simulink model "homeMobileManipulator"  (R2026a)
settings: Solver=ode4  StartTime=0  StopTime=Inf  FixedStep=cfg.rates.plant  MaxStep=cfg.rates.plant  AbsTol=1e-8
PostLoadFcn:
  | hmmSetup;
InitFcn:
  | hmmInitializeRun(bdroot);
values from neighbouring files (symbols this model uses):
  armJointLimits = zeros(numel(idx.arm), 2)    [hmmSetup.m]
  cfg = app.RunCfg    [HomeMobileManipulatorApp.m]    (also in HomeMobileManipulatorExample.m = params.cfg; hmmSetup.m = hmmConfig(); setupParams.m = data.cfg)
undefined symbols (not defined in the file or in its folder): actionQueueInit, actorNameTable, Angle, apertureMap, armPlanInit, Axis, basePlanInit, Custom, Extent, gray, gripperCoupling, invalidRayHits, movableRegistry, objectTargetInit, perceptionStatusInit, placeTargetInit, Position, robotStateInit, Sim3dSensor
libraries: robotmaniplib x20, robotcorelib x18, simulink x9, sim3dcameralib x6, sim3dgroundtruthsensorlib x4, dspmtrx3 x3, slpidlib x3, sim3dlib x3, hdlsllib x2, robotsim3dlib x1
(part 2 of 6)

== system homeMobileManipulator/Perception/GraspRefinement ==
  CameraFrames : Inport
  TaskRequest : Inport  Port=2
  ObjectTarget : Inport  Port=3
  RobotState : Inport  Port=4
  RefineRequestId : Inport  Port=5
  Refine : TriggerPort  VariantControl=(inherit)  PortDimensions=1
  CoarseTarget : BusSelector  OutputSignals=Position,Extent
  RefineService : MATLAB Function  TreatAsAtomicUnit=on
  SimTime : BusSelector  OutputSignals=Timestamp
  RefinedPosition : Outport
  RefineValid : Outport  Port=2
  RefineStatus : Outport  Port=3
  RefineShift : Outport  Port=4
  ServedRefineId : Outport  Port=5
  RefinedExtent : Outport  Description=THE EXTENT THE DESCENT SHOULD USE: the coarse extent with element 3 replaced by the height THIS FRAME MEASURED, and the coarse extent unchanged on every path that measured nothing. The same depth frame that locates the object top face also reads the support plane under it, so their difference is the object height - measured, with no manifest entry and no assumption. ONLY ELEMENT 3 MOVES, AND THE OTHER TWO ARE NOT A DEFECT WAITING TO BE FIXED: the horizontal extents drive the held-object collision box width and the jaw-aperture gate, and this look measures a top-face plateau, which is not the object silhouette. The height is different - the plateau rise above the support plane IS the height, for any shape. Resolved to a full extent inside hmmRefineService rather than here, so the diagram never has to test a magnitude and a zeros(3,1) can never reach a collision box or a grasp clamp.  Port=6
  wires:
  RefineService/6(RefinedExtent) -> RefinedExtent/1
  RefineService/5(ServedRefineId) -> ServedRefineId/1
  RefineService/4(RefineShift) -> RefineShift/1
  RefineService/2(RefineValid) -> RefineValid/1
  RefineService/1(RefinedPosition) -> RefinedPosition/1
  SimTime/1 -> RefineService/6(simTime)  "<Timestamp>"
  RefineRequestId/1 -> RefineService/5(requestId)
  CoarseTarget/1 -> RefineService/3(coarsePosition)  "<Position>"
  CameraFrames/1 -> RefineService/1(frames)
  RobotState/1 -> SimTime/1
  RefineService/3(RefineStatus) -> RefineStatus/1
  CoarseTarget/2 -> RefineService/4(coarseExtent)  "<Extent>"
  ObjectTarget/1 -> CoarseTarget/1
  TaskRequest/1 -> RefineService/2(task)

== system homeMobileManipulator/Perception/RefinementSelect ==
  ObjectTarget : Inport
  RefineRequestId : Inport  Port=2
  RefinedPosition : Inport  Port=3
  RefineValid : Inport  Port=4
  ServedRefineId : Inport  Port=5
  RefinedExtent : Inport  Port=6
  CoarseGraspPoint : BusSelector  Description=THE FALLBACK ARM OF THE REFINEMENT MERGE. Selects Position alone out of the COARSE ObjectTarget bus, the one Perception reconstructed from the four room cameras, and hands it to RefinedOrCoarse as the value to use when the wrist never got a usable second look. A BusSelector rather than tapping the bus twice downstream because the Switch needs a bare [3 1], and selecting here keeps the coarse-vs-refined choice visible as one three-block chain at root instead of hiding it inside a subsystem.  OutputSignals=Position,Extent
  CurrentRefinementValid : Logic  AllPortsSameDT=off  OutDataTypeStr=boolean
  ObjectTargetRefined : BusAssignment  Description=PUBLISHES THE REFINED GRASP POINT AND THE MEASURED OBJECT SIZE. Assigns Position and Extent and nothing else, so Label, GraspExtent, ActorId and the failure fields stay exactly as Perception sourced them. The wrist refines WHERE the object is and HOW TALL it is, never WHAT it is. Extent joined Position here once the wrist look began measuring the object height from its own depth frame: the same frame that locates the top face reads the support plane under it, and the difference is the height, so MotionPlanning/TargetSelect can aim the jaws at a measured mid-height instead of at a fraction of a manifest entry - or, for an object the manifest does not describe, instead of a flat cfg.percep.extentAssumed guess. ONLY ELEMENT 3 OF THE EXTENT EVER DIFFERS; the horizontal pair is passed through, because a top-face plateau is not the object silhouette. Feeds Manipulator and Gripper, the two consumers that touch the object: the arm plan descends to this point and the capture gate measures from it. TaskPlanner DELIBERATELY KEEPS THE COARSE BUS from Perception instead. It uses Position to form BaseGoalPose, which is solved before the base has driven anywhere and therefore long before the wrist has ever seen the object, so feeding it a point that does not exist yet would be an anachronism, not an improvement. The output signal is named ObjectTargetRefined and logged: hmmRunSummary resolves logged buses BY SIGNAL NAME, so leaving it unnamed made every report, plot and app view show the coarse point while the arm correctly flew to the refined one - a reader scoring the run against the report concluded the second look did nothing.  AssignedSignals=Position,Extent
  RefineRequestMatches : RelationalOperator  Operator===  OutDataTypeStr=boolean  RndMeth=Simplest  InputSameDT=off
  RefinedOrCoarse : Switch  Description=THE WRIST REFINEMENT IS ADVISORY, AND THIS BLOCK IS THE WHOLE REASON IT CAN BE. hmmWristRefine returns the coarse position UNCHANGED on every path that is not STATUS_APPLIED - no frame, no depth, out of range, no top face, a shift past cfg.refine.maxShift - and signals that by clearing RefineValid rather than by returning zeros. So u2 ~= 0 selects the refined point and anything else falls through to the coarse one. Without this switch a failed second look would drive the arm at the origin, which is strictly worse than never looking twice. MEASURED: on the shipped run the refined point cuts the lateral error at the mug body axis from 40.09 mm to 0.99 mm, so the APPLIED branch is worth having and the guarded fallback is what makes it safe to take.  Criteria=u2 ~= 0  SaturateOnIntegerOverflow=off  InputSameDT=off
  RefinedOrCoarseExtent : Switch  Description=THE SECOND ARM OF THE REFINEMENT MERGE, AND IT CARRIES A MEASUREMENT RATHER THAN A CORRECTION. RefinedOrCoarse next door chooses WHERE the object is; this one chooses WHAT SIZE it is. Takes the wrist-measured Extent when RefineValid, the coarse Extent otherwise. The two Switches are deliberately separate blocks on the same gate rather than one wider Switch, because the signals have different widths and because a reader should be able to see that a refinement either replaces both or replaces neither. Gated on RefineValid alone here, the height-is-positive condition having already been applied inside hmmRefineService - so this Switch never has to test a magnitude, and a zero-height Extent cannot reach a collision box or a grasp clamp by way of a sign error in the diagram.  Criteria=u2 ~= 0  SaturateOnIntegerOverflow=off  InputSameDT=off
  ObjectTargetInUse : Outport
  wires:
  ObjectTarget/1 -> ObjectTargetRefined/1, CoarseGraspPoint/1
  RefineRequestId/1 -> RefineRequestMatches/1
  ServedRefineId/1 -> RefineRequestMatches/2
  CoarseGraspPoint/2 -> RefinedOrCoarseExtent/3  "<Extent>"
  RefinedExtent/1 -> RefinedOrCoarseExtent/1
  CurrentRefinementValid/1 -> RefinedOrCoarseExtent/2, RefinedOrCoarse/2  "CurrentRefinementValid"
  RefineRequestMatches/1 -> CurrentRefinementValid/1  "RefineRequestMatches"
  RefineValid/1 -> CurrentRefinementValid/2
  RefinedPosition/1 -> RefinedOrCoarse/1
  CoarseGraspPoint/1 -> RefinedOrCoarse/3  "<Position>"
  RefinedOrCoarse/1 -> ObjectTargetRefined/2
  RefinedOrCoarseExtent/1 -> ObjectTargetRefined/3
  ObjectTargetRefined/1 -> ObjectTargetInUse/1  "ObjectTargetRefined"

== system homeMobileManipulator/Perception/SceneGrounding ==
  CameraFrames : Inport  OutDataTypeStr=Bus: CameraFrame  PortDimensions=5  LatchByDelayingOutsideSignal=on
  TaskRequest : Inport  Port=2  OutDataTypeStr=Bus: TaskRequest  LatchByDelayingOutsideSignal=on
  RobotState : Inport  Port=3  OutDataTypeStr=Bus: RobotState  LatchByDelayingOutsideSignal=on
  MovableRegistry : Inport  Port=4  OutDataTypeStr=Bus: MovableRegistry  LatchByDelayingOutsideSignal=on
  ActiveIndex : Inport  Description=Latch the selected queue index before the perception trigger to break planner feedback. The existing capture delay allows the index to settle before reconstruction.  Port=5  OutDataTypeStr=uint8  LatchByDelayingOutsideSignal=on
  Send : TriggerPort  VariantControl=Variant  PortDimensions=1
  Grounding : Subsystem
  Reconstruction : Subsystem
  SceneMapping : Subsystem
  SimTime : BusSelector  OutputSignals=Timestamp
  ActionQueue : Outport  OutDataTypeStr=Bus: ActionQueue  InitialOutput=actionQueueInit
  ObjectTarget : Outport  Port=2  OutDataTypeStr=Bus: ObjectTarget  InitialOutput=objectTargetInit
  PlaceTarget : Outport  Port=3  OutDataTypeStr=Bus: PlaceTarget  InitialOutput=placeTargetInit
  PerceptionStatus : Outport  Port=4  OutDataTypeStr=Bus: PerceptionStatus  InitialOutput=perceptionStatusInit
  wires:
  CameraFrames/1 -> SceneMapping/1(CameraFrames), Reconstruction/1(CameraFrames), Grounding/1(CameraFrames)
  Grounding/2(PerceptionStatus) -> PerceptionStatus/1
  RobotState/1 -> SceneMapping/2(RobotState), SimTime/1
  TaskRequest/1 -> Grounding/2(TaskRequest)
  MovableRegistry/1 -> Reconstruction/3(MovableRegistry)
  ActiveIndex/1 -> Grounding/4(ActiveIndex)
  Grounding/1(ActionQueue) -> ActionQueue/1, Reconstruction/2(ActionQueue)
  SimTime/1 -> Reconstruction/4(SimTime), Grounding/3(SimTime)  "<Timestamp>"
  Reconstruction/1(ObjectTarget) -> ObjectTarget/1
  Reconstruction/2(PlaceTarget) -> PlaceTarget/1

== system homeMobileManipulator/MobileManipulator/Gripper/ClosureDetect ==
  ApertureCmd : Inport
  Aperture : Inport  Port=2
  DriverAngle : Inport  Port=3
  AbsError : Abs
  ApertureError : Sum  Inputs=+-
  ApertureTol : Constant  Value=cfg.gripper.apertureTol
  AtCommand : RelationalOperator  Operator=<=  OutDataTypeStr=boolean  InputSameDT=off
  DriverMoving : simulink/Logic and Bit Operations/Detect Change  vinit=0  OutDataTypeStr=boolean
      settings: LibrarySourceBlock=|
      | hdlsllib/Logic and Bit
      | Operations/Detect
      | Change
  DriverStopped : Logic  Operator=NOT  IconShape=distinctive  AllPortsSameDT=off  OutDataTypeStr=boolean
  SettledAnd : Logic  IconShape=distinctive  AllPortsSameDT=off  OutDataTypeStr=boolean
  Settled : Outport
  wires:
  DriverStopped/1 -> SettledAnd/2  "DriverStopped"
  ApertureError/1 -> AbsError/1  "ApertureError"
  SettledAnd/1 -> Settled/1
  AbsError/1 -> AtCommand/1  "AbsError"
  ApertureTol/1 -> AtCommand/2
  DriverMoving/1 -> DriverStopped/1
  AtCommand/1 -> SettledAnd/1  "AtCommand"
  ApertureCmd/1 -> ApertureError/1
  Aperture/1 -> ApertureError/2
  DriverAngle/1 -> DriverMoving/1

== system homeMobileManipulator/MobileManipulator/Gripper/GraspCandidate ==
  ObjectTarget : Inport  OutDataTypeStr=Bus: ObjectTarget
  CloseRequested : Inport  Port=2
  ActorSelect : Switch  Criteria=u2 ~= 0
  Candidate : BusCreator  Inputs=5  OutDataTypeStr=Bus: GraspCandidate  NonVirtualBus=on
      settings: InheritFromInputs=off
  CandidateValid : Logic  IconShape=distinctive  AllPortsSameDT=off  OutDataTypeStr=boolean
  HalfHeight : Gain  Description=THE CAPTURE GATE MEASURES TO THE OBJECT'S CENTRE, AND ObjectTarget.Position IS NOT IT. Position is the SUPPORT SURFACE under the object - see the Position contract in hmmReconstructTargets and hmmDefineBuses - so half the sourced height, Extent(3)/2, is what carries it to the centre. A matrix gain rather than a Selector and a scalar gain because the result has to be a [3 1] the Sum below can add to Position without a second reshape: [0 0 0; 0 0 0; 0 0 0.5] annihilates x and y and halves z in one block.  Gain=[0 0 0; 0 0 0; 0 0 0.5]  Multiplication=Matrix(K*u)
  NoActor : Constant  Value=cfg.actor.noneId  OutDataTypeStr=uint8  SampleTime=-1
  ObjSelect : BusSelector  OutputSignals=ActorId,Position,GraspExtent,NumCandidates,Valid,Extent
  ObjectCentre : Sum  Description=WHY THE CENTRE AND NOT THE POINT THE ARM WAS AIMED AT. cfg.grasp.captureRadius is cfg.gripper.maxOpenPos/2 + cfg.grasp.captureMargin - the half jaw stroke plus a margin - so it is a statement about the OBJECT lying inside the volume the jaws sweep, not about how well the servo tracked. Comparing the grasp frame against the commanded grasp point instead would reduce the gate to a tracking check that TrackingMetrics already performs, and would make it blind to the one error it exists to catch. WHAT THIS FIXED. Position was fed to GraspCandidate verbatim, so once the Position contract became the support surface the whole deliberate grasp rise - cfg.grasp.heightFraction*Extent(3) + padDrop(GraspExtent), 66.0 mm on the shipped mug - was charged to the gate as error. WithinCapture measured 66.1 mm against a 62.5 mm radius, InCapture went false, and the close faulted NotGraspable with the tool 0.1 mm from the refined target in xy. It had been passing only because the tool used to sit BELOW the support surface (-16.8 mm on the reference run), which is the defect the grasp-height work removed. WHAT IT COSTS. The gate now spends (heightFraction - 1/2)*Extent(3) + padDrop on the deliberate offset: 21.1 mm for the mug, 39.9 mm for the Bottle, the tallest prop that survives the GraspExtent gate. That leaves 58.8 mm and 48.1 mm of horizontal budget respectively, against a 0.1 mm measured tracking error.
  GraspCandidate : Outport  OutDataTypeStr=Bus: GraspCandidate
  wires:
  ActorSelect/1 -> Candidate/1
  HalfHeight/1 -> ObjectCentre/2  "HalfHeight"
  Candidate/1 -> GraspCandidate/1
  ObjSelect/1 -> ActorSelect/1  "<ActorId>"
  ObjSelect/2 -> ObjectCentre/1  "<Position>"
  ObjectCentre/1 -> Candidate/2  "Position"
  ObjSelect/3 -> Candidate/3  "<GraspExtent>"
  ObjSelect/4 -> Candidate/4  "<NumCandidates>"
  ObjSelect/5 -> CandidateValid/1  "<Valid>"
  ObjSelect/6 -> HalfHeight/1  "<Extent>"
  NoActor/1 -> ActorSelect/3
  ObjectTarget/1 -> ObjSelect/1
  CloseRequested/1 -> CandidateValid/2
  CandidateValid/1 -> ActorSelect/2, Candidate/5  "Valid"

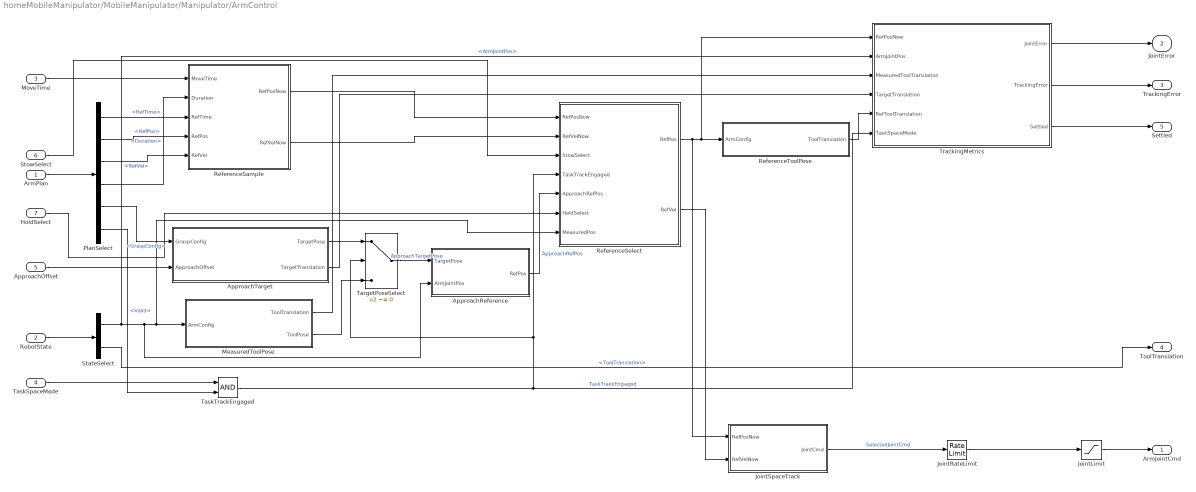
== system homeMobileManipulator/MobileManipulator/Manipulator/ArmControl ==
  ArmPlan : Inport
  RobotState : Inport  Port=2
  MoveTime : Inport  Port=3
  TaskSpaceMode : Inport  Port=4
  ApproachOffset : Inport  Port=5
  StowSelect : Inport  Port=6
  HoldSelect : Inport  Port=7
  ApproachReference : Subsystem  Description=|
      | The joint REFERENCE for a constrained approach or retreat, solved by inverse kinematics that is SEEDED WITH THE MEASURED CONFIGURATION.
      | 
      | WHY THIS EXISTS, AND WHAT IT REPLACES. ArmControl used to carry a second tracker - a Task Space Motion Model - and ModeSelect switched the joint COMMAND between it and JointSpaceTrack on TaskTrackEngaged. Both motion models integrate their own configuration from cfg.arm.stowConfig at t = 0, always, and nothing ever reconciled them. Feeding the task-space model the MEASURED TOOL POSE while it was disengaged was an attempt at bumpless transfer, and it cannot work: a tool pose does not determine a configuration. Measured on the 20 s run, the task-space model free-ran for 6.8 s and settled on a different IK branch - elbow sign-flipped and wrist-3 off by very nearly pi - 4.467 rad from where the arm actually was. ModeSelect handed that branch to JointRateLimit, which ramped toward it at cfg.arm.jointVelMax, the tool error passed cfg.safety.trackErrMax 0.15 s later, and Retreating's tracking guard reported ArmPlanFailed for a plan that had been tracked to 3.4 mm.
      | 
      | SO THERE IS NOW ONE INTEGRATOR. JointSpaceTrack is the only tracker; approach and retreat produce a REFERENCE for it instead of a competing command. TargetPoseSelect is kept and still feeds the approach target when engaged and the measured tool pose when not, but it now feeds an IK solve rather than a motion model - and THE SEED IS WHAT MAKES THAT SOUND. Seeding with the measured configuration pins the solution to the branch the arm is already on, so at the instant of engagement the target is the grasp pose at zero offset, the seed is the current configuration, and the answer is the current configuration. Continuity is a property of the construction rather than something to be hoped for.
  ApproachTarget : Subsystem
  JointLimit : Saturate  UpperLimit=armJointLimits(:,2)  LowerLimit=armJointLimits(:,1)
  JointRateLimit : RateLimiter  RisingSlewLimit=cfg.arm.jointVelMax'  FallingSlewLimit=-cfg.arm.jointVelMax'  SampleTimeMode=inherited  InitialCondition=cfg.arm.stowConfig'
  JointSpaceTrack : Subsystem
  MeasuredToolPose : Subsystem
  PlanSelect : BusSelector  OutputSignals=RefTime,RefPos,RefVel,Duration,GraspConfig,Valid
  ReferenceSample : Subsystem
  ReferenceSelect : Subsystem
  ReferenceToolPose : Subsystem
  StateSelect : BusSelector  OutputSignals=ArmJointPos,ToolTranslation
  TargetPoseSelect : Switch  Description=|  Criteria=u2 ~= 0
      | Approach target when engaged, measured tool pose when not.
      | 
      | Kept from the design this replaces, because the intent was right: the branch that is not in control must be commanded to where the arm IS, so that engaging it is not a step. What changed is the consumer. Handing this to a Task Space Motion Model did not work, because that block integrates its own configuration and a pose does not determine one. Handing it to an IK solve seeded with the measured configuration does.
  TaskTrackEngaged : Logic  Description=The task-space tracker is engaged only when the supervisor asks for task-space mode AND the plan it would chase is valid. Both halves are load-bearing. Without the mode term the tracker integrates through every phase of the task; without the Valid term it chases a GraspConfig that is all zeros when planning failed, which for a UR5e is the fully outstretched singular pose, and the operational-space gains are meaningless there.  AllPortsSameDT=off  OutDataTypeStr=boolean
  TrackingMetrics : Subsystem
  ArmJointCmd : Outport
  JointError : Outport  Port=2
  TrackingError : Outport  Port=3
  ToolTranslation : Outport  Port=4
  Settled : Outport  Port=5
  wires:
  JointRateLimit/1 -> JointLimit/1
  TrackingMetrics/2(TrackingError) -> TrackingError/1
  TrackingMetrics/1(JointError) -> JointError/1
  JointSpaceTrack/1(JointCmd) -> JointRateLimit/1  "SelectedJointCmd"
  ReferenceSelect/2(RefVel) -> JointSpaceTrack/2(RefVelNow)
  ReferenceSelect/1(RefPos) -> ReferenceToolPose/1(ArmConfig), TrackingMetrics/1(RefPosNow), JointSpaceTrack/1(RefPosNow)
  HoldSelect/1 -> ReferenceSelect/6(HoldSelect)
  ApproachReference/1(RefPos) -> ReferenceSelect/5(ApproachRefPos)  "ApproachRefPos"
  TargetPoseSelect/1 -> ApproachReference/1(TargetPose)  "ApproachTargetPose"
  MeasuredToolPose/2(ToolPose) -> TargetPoseSelect/3
  MeasuredToolPose/1(ToolTranslation) -> TrackingMetrics/3(MeasuredToolTranslation)
  ApproachTarget/2(TargetTranslation) -> TrackingMetrics/4(TargetTranslation)
  ApproachTarget/1(TargetPose) -> TargetPoseSelect/1
  ReferenceSample/2(RefVelNow) -> ReferenceSelect/2(RefVelNow)
  ReferenceSample/1(RefPosNow) -> ReferenceSelect/1(RefPosNow)
  TaskSpaceMode/1 -> TaskTrackEngaged/1
  StateSelect/2 -> ToolTranslation/1  "<ToolTranslation>"
  StateSelect/1 -> MeasuredToolPose/1(ArmConfig), ReferenceSelect/7(MeasuredPos), ApproachReference/2(ArmJointPos), TrackingMetrics/2(ArmJointPos)  "<ArmJointPos>"
  JointLimit/1 -> ArmJointCmd/1
  PlanSelect/6 -> TaskTrackEngaged/2  "<Valid>"
  ReferenceToolPose/1(ToolTranslation) -> TrackingMetrics/5(RefToolTranslation)
  TrackingMetrics/3(Settled) -> Settled/1
  PlanSelect/4 -> ReferenceSample/2(Duration)  "<Duration>"
  TaskTrackEngaged/1 -> ReferenceSelect/4(TaskTrackEngaged), TargetPoseSelect/2, TrackingMetrics/6(TaskSpaceMode)  "TaskTrackEngaged"
  PlanSelect/3 -> ReferenceSample/5(RefVel)  "<RefVel>"
  PlanSelect/2 -> ReferenceSample/4(RefPos)  "<RefPos>"
  PlanSelect/1 -> ReferenceSample/3(RefTime)  "<RefTime>"
  PlanSelect/5 -> ApproachTarget/1(GraspConfig)  "<GraspConfig>"
  ArmPlan/1 -> PlanSelect/1
  ApproachOffset/1 -> ApproachTarget/2(ApproachOffset)
  RobotState/1 -> StateSelect/1
  StowSelect/1 -> ReferenceSelect/3(StowSelect)
  MoveTime/1 -> ReferenceSample/1(MoveTime)

== system homeMobileManipulator/MobileManipulator/Manipulator/MotionPlanning ==
  RequestId : Inport  OutDataTypeStr=uint32
  ObjectTarget : Inport  Port=2  OutDataTypeStr=Bus: ObjectTarget
  PlaceTarget : Inport  Port=3  OutDataTypeStr=Bus: PlaceTarget
  RobotState : Inport  Port=4  OutDataTypeStr=Bus: RobotState
  ArmMode : Inport  Port=5  OutDataTypeStr=uint8
  Enable : EnablePort  StatesWhenEnabling=reset
  CandidateIK : Subsystem
  ConfigAssembly : Subsystem
  MapToArmFrame : robotmaniplib/Get Transform  RigidBodyTree=robot  SourceBody=map  TargetBody=arm_mount  SimulateUsing=Code generation
  PrevPlan : UnitDelay  InitialCondition=armPlanInit  SampleTime=-1
  ScreenAndPlan : MATLAB Function  Description=SIMULINK-FIRST JUSTIFICATION: no block in any installed library screens grasp candidates, searches with manipulatorRRT and parameterises with contopptraj. (a) No dedicated toolbox block: find_system('robotmaniplib','SearchDepth',2,'Type','Block') returns 10 blocks - Forward Dynamics, Get Jacobian, Get Transform, Gravity Torque, Inverse Dynamics, Inverse Kinematics, Joint Space Mass Matrix, Joint Space Motion Model, Task Space Motion Model, Velocity Product Torque - and not one of them is a path planner, a collision checker or a time-optimal parameteriser. The four that DO cover part of this job are used as blocks: three Inverse Kinematics, three Get Jacobian, one Get Transform, three Reciprocal Condition. (b) No native Simulink equivalent: manipulatorRRT, checkCollision and contopptraj have no primitive composition - a sampling-based tree search is not a block diagram. (c) The native equivalent is not merely over 15 blocks, it does not exist. Called through coder.extrinsic; the model stays in normal mode.  TreatAsAtomicUnit=on
  SimTime : BusSelector  OutputSignals=Timestamp
  TargetSelect : Subsystem
  ArmPlan : Outport  OutDataTypeStr=Bus: ArmPlan  InitialOutput=armPlanInit
  wires:
  PrevPlan/1 -> ScreenAndPlan/12(planTemplate)
  RequestId/1 -> ScreenAndPlan/10(requestId)
  ScreenAndPlan/1(aplan) -> ArmPlan/1, PrevPlan/1
  CandidateIK/4(GraspPoses) -> ScreenAndPlan/9(graspPoses)
  CandidateIK/3(Manipulability) -> ScreenAndPlan/8(manipulability)
  CandidateIK/2(PoseErrors) -> ScreenAndPlan/7(poseErrors)
  CandidateIK/1(GraspConfigs) -> ScreenAndPlan/6(graspConfigs)
  SimTime/1 -> ScreenAndPlan/11(simTime)  "<Timestamp>"
  MapToArmFrame/1 -> CandidateIK/2(TfArmFromMap), ScreenAndPlan/5(tfArmFromMap)
  ConfigAssembly/2(IkGuess) -> CandidateIK/3(IkGuess)
  ConfigAssembly/1(RobotConfig) -> MapToArmFrame/1, ScreenAndPlan/4(robotConfig)
  PlaceTarget/1 -> TargetSelect/2(PlaceTarget), ScreenAndPlan/2(placeTarget)
  ArmMode/1 -> ScreenAndPlan/3(mode), TargetSelect/3(ArmMode)
  RobotState/1 -> ConfigAssembly/1(RobotState), SimTime/1
  ObjectTarget/1 -> TargetSelect/1(ObjectTarget), ScreenAndPlan/1(objectTarget)
  TargetSelect/1(GraspPoint) -> CandidateIK/1(GraspPoint)

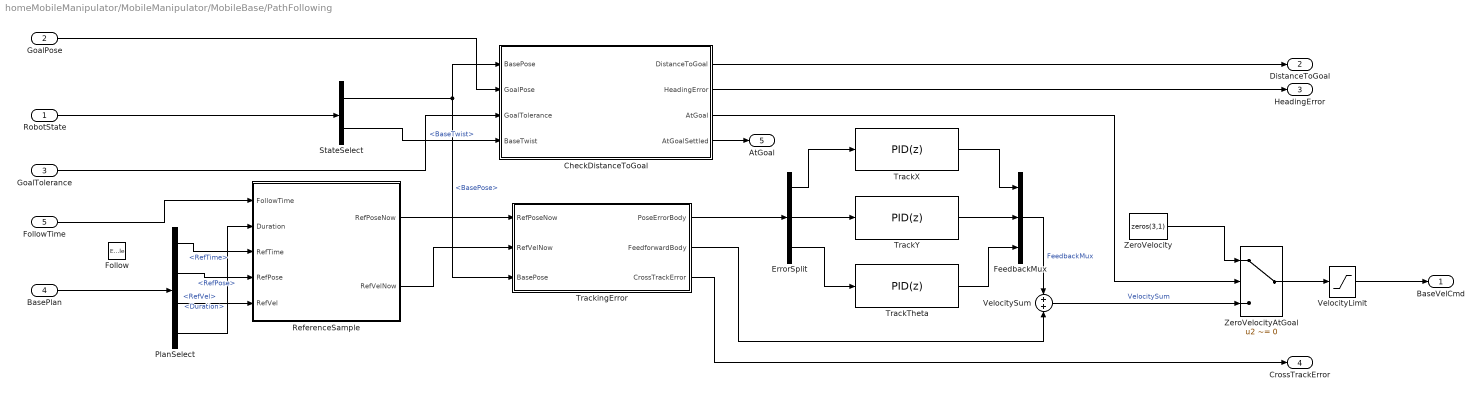
== system homeMobileManipulator/MobileManipulator/MobileBase/PathFollowing ==
  RobotState : Inport
  GoalPose : Inport  Port=2
  GoalTolerance : Inport  Port=3
  BasePlan : Inport  Port=4
  FollowTime : Inport  Port=5
  Follow : EnablePort  StatesWhenEnabling=reset
  CheckDistanceToGoal : Subsystem
  ErrorSplit : Demux  Outputs=3
  FeedbackMux : Mux  Inputs=3
  PlanSelect : BusSelector  OutputSignals=RefTime,RefPose,RefVel,Duration
  ReferenceSample : Subsystem
  StateSelect : BusSelector  OutputSignals=BasePose,BaseTwist
  TrackTheta : slpidlib/PID Controller  Controller=PID  Form=Parallel  TimeDomain=Discrete-time  UseExternalTs=off  SampleTime=cfg.rates.control  IntegratorMethod=Trapezoidal  FilterMethod=Forward Euler  ControllerParametersSource=internal  P=cfg.track.kpTheta  I=cfg.track.kiTheta  UseKiTs=off  D=cfg.track.kdTheta  UseExternalDerivativeSource=off  N=100  UseFilter=on  TunerSelectOption=Transfer Function Based (PID Tuner App)  InitialConditionSource=internal  InitialConditionForIntegrator=0  InitialConditionForFilter=0  DifferentiatorICPrevScaledInput=0  ExternalReset=none  TrackingMode=off  Kt=1  LimitOutput=on  SatLimitsSource=internal  UpperSaturationLimit=cfg.base.omegaMax  LowerSaturationLimit=-cfg.base.omegaMax  LinearizeAsGain=off  AntiWindupMode=clamping  Kb=1  LimitIntegrator=off  UpperIntegratorSaturationLimit=inf  LowerIntegratorSaturationLimit=-inf  POutMin=[]  POutMax=[]  IOutMin=[]  IOutMax=[]  DOutMin=[]  DOutMax=[]  NOutMin=[]  NOutMax=[]  SumOutMin=[]  SumOutMax=[]  SaturationOutMin=[]  SaturationOutMax=[]  PParamMin=[]  PParamMax=[]  IParamMin=[]  IParamMax=[]  DParamMin=[]  DParamMax=[]  NParamMin=[]  NParamMax=[]  KbParamMin=[]  KbParamMax=[]  KtParamMin=[]  KtParamMax=[]  KbOutMin=[]  KbOutMax=[]  KtOutMin=[]  KtOutMax=[]  IntegratorOutMin=[]  IntegratorOutMax=[]  FilterOutMin=[]  FilterOutMax=[]  SumI1OutMin=[]  SumI1OutMax=[]  SumI2OutMin=[]  SumI2OutMax=[]  SumI3OutMin=[]  SumI3OutMax=[]  SumI4OutMin=[]  SumI4OutMax=[]  SumDOutMin=[]  SumDOutMax=[]  DifferentiatorOutMin=[]  DifferentiatorOutMax=[]  FilterDiffOutCoefMin=[]  FilterDiffOutCoefMax=[]  ReciprocalOutMin=[]  ReciprocalOutMax=[]  SumDenOutMin=[]  SumDenOutMax=[]  SumNumOutMin=[]  SumNumOutMax=[]  DivideOutMin=[]  DivideOutMax=[]  UdiffTsProdOutMin=[]  UdiffTsProdOutMax=[]  NTsProdOutMin=[]  NTsProdOutMax=[]  UintegralTsProdOutMin=[]  UintegralTsProdOutMax=[]  UngainTsProdOutMin=[]  UngainTsProdOutMax=[]  ClampingZeroOutDataTypeStr=Inherit: Inherit via back propagation  ClampingZeroOutMin=[]  ClampingZeroOutMax=[]  FilterDenConstantOutDataTypeStr=Inherit: Inherit via back propagation  FilterDenConstantOutMin=[]  FilterDenConstantOutMax=[]  PCopyOutDataTypeStr=Inherit: Inherit via back propagation  PCopyOutMin=[]  PCopyOutMax=[]  NCopyOutDataTypeStr=Inherit: Inherit via back propagation  NCopyOutMin=[]  NCopyOutMax=[]  IntegratorContinuousStateAttributes=''  IntegratorStateMustResolveToSignalObject=off  IntegratorRTWStateStorageClass=Auto  FilterContinuousStateAttributes=''  FilterStateMustResolveToSignalObject=off  FilterRTWStateStorageClass=Auto  ParallelPVariant=InternalParameters  IdealPVariant=Disabled  IVariant=InternalParameters  DVariant=InternalParameters  IntegratorVariant=Discrete  SatVariant=Enabled  AWVariant=DiscClampingParallel  PCopyVariant=Disabled  TRVariant=Disabled  FdbkBlocksVariant=Feedback  IdealPFdbkVariant=Passthrough  SatFdbkVariant=Passthrough  DerivativeFilterVariant=ForwardEulerFilter  NVariant=InternalParameters  NCopyVariant=Disabled  FilterICVariant=InternalICsFilter  IntegratorICVariant=InternalICs  ExternalResetVariant=Disabled  TRSumVariant=Passthrough  SumFdbkVariant=Enabled  SumVariant=Sum_PID  TsampFilterVariant=InternalTs  TsampNgainVariant=Passthrough  TsampIntegralVariant=Disabled_SignalSpec  ExternalSaturationOutDataTypeStr=Inherit: Same as second input  DerivativeSourceVariant=ErrorSignal  PreIntVariant=InternalPreInt
      settings: LibrarySourceBlock=simulink/Discrete/Discrete PID Controller
  TrackX : slpidlib/PID Controller  Controller=PID  Form=Parallel  TimeDomain=Discrete-time  UseExternalTs=off  SampleTime=cfg.rates.control  IntegratorMethod=Trapezoidal  FilterMethod=Forward Euler  ControllerParametersSource=internal  P=cfg.track.kpXY  I=cfg.track.kiXY  UseKiTs=off  D=cfg.track.kdXY  UseExternalDerivativeSource=off  N=100  UseFilter=on  TunerSelectOption=Transfer Function Based (PID Tuner App)  InitialConditionSource=internal  InitialConditionForIntegrator=0  InitialConditionForFilter=0  DifferentiatorICPrevScaledInput=0  ExternalReset=none  TrackingMode=off  Kt=1  LimitOutput=on  SatLimitsSource=internal  UpperSaturationLimit=cfg.base.vxMax  LowerSaturationLimit=-cfg.base.vxMax  LinearizeAsGain=off  AntiWindupMode=clamping  Kb=1  LimitIntegrator=off  UpperIntegratorSaturationLimit=inf  LowerIntegratorSaturationLimit=-inf  POutMin=[]  POutMax=[]  IOutMin=[]  IOutMax=[]  DOutMin=[]  DOutMax=[]  NOutMin=[]  NOutMax=[]  SumOutMin=[]  SumOutMax=[]  SaturationOutMin=[]  SaturationOutMax=[]  PParamMin=[]  PParamMax=[]  IParamMin=[]  IParamMax=[]  DParamMin=[]  DParamMax=[]  NParamMin=[]  NParamMax=[]  KbParamMin=[]  KbParamMax=[]  KtParamMin=[]  KtParamMax=[]  KbOutMin=[]  KbOutMax=[]  KtOutMin=[]  KtOutMax=[]  IntegratorOutMin=[]  IntegratorOutMax=[]  FilterOutMin=[]  FilterOutMax=[]  SumI1OutMin=[]  SumI1OutMax=[]  SumI2OutMin=[]  SumI2OutMax=[]  SumI3OutMin=[]  SumI3OutMax=[]  SumI4OutMin=[]  SumI4OutMax=[]  SumDOutMin=[]  SumDOutMax=[]  DifferentiatorOutMin=[]  DifferentiatorOutMax=[]  FilterDiffOutCoefMin=[]  FilterDiffOutCoefMax=[]  ReciprocalOutMin=[]  ReciprocalOutMax=[]  SumDenOutMin=[]  SumDenOutMax=[]  SumNumOutMin=[]  SumNumOutMax=[]  DivideOutMin=[]  DivideOutMax=[]  UdiffTsProdOutMin=[]  UdiffTsProdOutMax=[]  NTsProdOutMin=[]  NTsProdOutMax=[]  UintegralTsProdOutMin=[]  UintegralTsProdOutMax=[]  UngainTsProdOutMin=[]  UngainTsProdOutMax=[]  ClampingZeroOutDataTypeStr=Inherit: Inherit via back propagation  ClampingZeroOutMin=[]  ClampingZeroOutMax=[]  FilterDenConstantOutDataTypeStr=Inherit: Inherit via back propagation  FilterDenConstantOutMin=[]  FilterDenConstantOutMax=[]  PCopyOutDataTypeStr=Inherit: Inherit via back propagation  PCopyOutMin=[]  PCopyOutMax=[]  NCopyOutDataTypeStr=Inherit: Inherit via back propagation  NCopyOutMin=[]  NCopyOutMax=[]  IntegratorContinuousStateAttributes=''  IntegratorStateMustResolveToSignalObject=off  IntegratorRTWStateStorageClass=Auto  FilterContinuousStateAttributes=''  FilterStateMustResolveToSignalObject=off  FilterRTWStateStorageClass=Auto  ParallelPVariant=InternalParameters  IdealPVariant=Disabled  IVariant=InternalParameters  DVariant=InternalParameters  IntegratorVariant=Discrete  SatVariant=Enabled  AWVariant=DiscClampingParallel  PCopyVariant=Disabled  TRVariant=Disabled  FdbkBlocksVariant=Feedback  IdealPFdbkVariant=Passthrough  SatFdbkVariant=Passthrough  DerivativeFilterVariant=ForwardEulerFilter  NVariant=InternalParameters  NCopyVariant=Disabled  FilterICVariant=InternalICsFilter  IntegratorICVariant=InternalICs  ExternalResetVariant=Disabled  TRSumVariant=Passthrough  SumFdbkVariant=Enabled  SumVariant=Sum_PID  TsampFilterVariant=InternalTs  TsampNgainVariant=Passthrough  TsampIntegralVariant=Disabled_SignalSpec  ExternalSaturationOutDataTypeStr=Inherit: Same as second input  DerivativeSourceVariant=ErrorSignal  PreIntVariant=InternalPreInt
      settings: LibrarySourceBlock=simulink/Discrete/Discrete PID Controller
  TrackY : slpidlib/PID Controller  Controller=PID  Form=Parallel  TimeDomain=Discrete-time  UseExternalTs=off  SampleTime=cfg.rates.control  IntegratorMethod=Trapezoidal  FilterMethod=Forward Euler  ControllerParametersSource=internal  P=cfg.track.kpXY  I=cfg.track.kiXY  UseKiTs=off  D=cfg.track.kdXY  UseExternalDerivativeSource=off  N=100  UseFilter=on  TunerSelectOption=Transfer Function Based (PID Tuner App)  InitialConditionSource=internal  InitialConditionForIntegrator=0  InitialConditionForFilter=0  DifferentiatorICPrevScaledInput=0  ExternalReset=none  TrackingMode=off  Kt=1  LimitOutput=on  SatLimitsSource=internal  UpperSaturationLimit=cfg.base.vyMax  LowerSaturationLimit=-cfg.base.vyMax  LinearizeAsGain=off  AntiWindupMode=clamping  Kb=1  LimitIntegrator=off  UpperIntegratorSaturationLimit=inf  LowerIntegratorSaturationLimit=-inf  POutMin=[]  POutMax=[]  IOutMin=[]  IOutMax=[]  DOutMin=[]  DOutMax=[]  NOutMin=[]  NOutMax=[]  SumOutMin=[]  SumOutMax=[]  SaturationOutMin=[]  SaturationOutMax=[]  PParamMin=[]  PParamMax=[]  IParamMin=[]  IParamMax=[]  DParamMin=[]  DParamMax=[]  NParamMin=[]  NParamMax=[]  KbParamMin=[]  KbParamMax=[]  KtParamMin=[]  KtParamMax=[]  KbOutMin=[]  KbOutMax=[]  KtOutMin=[]  KtOutMax=[]  IntegratorOutMin=[]  IntegratorOutMax=[]  FilterOutMin=[]  FilterOutMax=[]  SumI1OutMin=[]  SumI1OutMax=[]  SumI2OutMin=[]  SumI2OutMax=[]  SumI3OutMin=[]  SumI3OutMax=[]  SumI4OutMin=[]  SumI4OutMax=[]  SumDOutMin=[]  SumDOutMax=[]  DifferentiatorOutMin=[]  DifferentiatorOutMax=[]  FilterDiffOutCoefMin=[]  FilterDiffOutCoefMax=[]  ReciprocalOutMin=[]  ReciprocalOutMax=[]  SumDenOutMin=[]  SumDenOutMax=[]  SumNumOutMin=[]  SumNumOutMax=[]  DivideOutMin=[]  DivideOutMax=[]  UdiffTsProdOutMin=[]  UdiffTsProdOutMax=[]  NTsProdOutMin=[]  NTsProdOutMax=[]  UintegralTsProdOutMin=[]  UintegralTsProdOutMax=[]  UngainTsProdOutMin=[]  UngainTsProdOutMax=[]  ClampingZeroOutDataTypeStr=Inherit: Inherit via back propagation  ClampingZeroOutMin=[]  ClampingZeroOutMax=[]  FilterDenConstantOutDataTypeStr=Inherit: Inherit via back propagation  FilterDenConstantOutMin=[]  FilterDenConstantOutMax=[]  PCopyOutDataTypeStr=Inherit: Inherit via back propagation  PCopyOutMin=[]  PCopyOutMax=[]  NCopyOutDataTypeStr=Inherit: Inherit via back propagation  NCopyOutMin=[]  NCopyOutMax=[]  IntegratorContinuousStateAttributes=''  IntegratorStateMustResolveToSignalObject=off  IntegratorRTWStateStorageClass=Auto  FilterContinuousStateAttributes=''  FilterStateMustResolveToSignalObject=off  FilterRTWStateStorageClass=Auto  ParallelPVariant=InternalParameters  IdealPVariant=Disabled  IVariant=InternalParameters  DVariant=InternalParameters  IntegratorVariant=Discrete  SatVariant=Enabled  AWVariant=DiscClampingParallel  PCopyVariant=Disabled  TRVariant=Disabled  FdbkBlocksVariant=Feedback  IdealPFdbkVariant=Passthrough  SatFdbkVariant=Passthrough  DerivativeFilterVariant=ForwardEulerFilter  NVariant=InternalParameters  NCopyVariant=Disabled  FilterICVariant=InternalICsFilter  IntegratorICVariant=InternalICs  ExternalResetVariant=Disabled  TRSumVariant=Passthrough  SumFdbkVariant=Enabled  SumVariant=Sum_PID  TsampFilterVariant=InternalTs  TsampNgainVariant=Passthrough  TsampIntegralVariant=Disabled_SignalSpec  ExternalSaturationOutDataTypeStr=Inherit: Same as second input  DerivativeSourceVariant=ErrorSignal  PreIntVariant=InternalPreInt
      settings: LibrarySourceBlock=simulink/Discrete/Discrete PID Controller
  TrackingError : Subsystem
  VelocityLimit : Saturate  UpperLimit=cfg.base.cmdMargin*[cfg.base.vxMax; cfg.base.vyMax; cfg.base.omegaMax]  LowerLimit=-cfg.base.cmdMargin*[cfg.base.vxMax; cfg.base.vyMax; cfg.base.omegaMax]
  VelocitySum : Sum
  ZeroVelocity : Constant  Value=zeros(3,1)
  ZeroVelocityAtGoal : Switch  Criteria=u2 ~= 0
  BaseVelCmd : Outport  OutputWhenDisabled=reset  InitialOutput=zeros(3,1)
  DistanceToGoal : Outport  Port=2  InitialOutput=0
  HeadingError : Outport  Port=3  InitialOutput=0
  CrossTrackError : Outport  Port=4  InitialOutput=0
  AtGoal : Outport  Port=5  OutputWhenDisabled=reset  InitialOutput=false
  wires:
  VelocityLimit/1 -> BaseVelCmd/1
  ZeroVelocityAtGoal/1 -> VelocityLimit/1
  ZeroVelocity/1 -> ZeroVelocityAtGoal/1
  TrackTheta/1 -> FeedbackMux/3
  TrackY/1 -> FeedbackMux/2
  TrackX/1 -> FeedbackMux/1
  ErrorSplit/3 -> TrackTheta/1
  TrackingError/1(PoseErrorBody) -> ErrorSplit/1
  ErrorSplit/1 -> TrackX/1
  FeedbackMux/1 -> VelocitySum/1  "FeedbackMux"
  CheckDistanceToGoal/4(AtGoalSettled) -> AtGoal/1
  CheckDistanceToGoal/3(AtGoal) -> ZeroVelocityAtGoal/2
  VelocitySum/1 -> ZeroVelocityAtGoal/3  "VelocitySum"
  CheckDistanceToGoal/2(HeadingError) -> HeadingError/1
  ReferenceSample/2(RefVelNow) -> TrackingError/2(RefVelNow)
  StateSelect/2 -> CheckDistanceToGoal/4(BaseTwist)  "<BaseTwist>"
  TrackingError/3(CrossTrackError) -> CrossTrackError/1
  StateSelect/1 -> TrackingError/3(BasePose), CheckDistanceToGoal/1(BasePose)  "<BasePose>"
  GoalTolerance/1 -> CheckDistanceToGoal/3(GoalTolerance)
  GoalPose/1 -> CheckDistanceToGoal/2(GoalPose)
  PlanSelect/3 -> ReferenceSample/5(RefVel)  "<RefVel>"
  ReferenceSample/1(RefPoseNow) -> TrackingError/1(RefPoseNow)
  PlanSelect/1 -> ReferenceSample/3(RefTime)  "<RefTime>"
  ErrorSplit/2 -> TrackY/1
  FollowTime/1 -> ReferenceSample/1(FollowTime)
  CheckDistanceToGoal/1(DistanceToGoal) -> DistanceToGoal/1
  TrackingError/2(FeedforwardBody) -> VelocitySum/2
  PlanSelect/4 -> ReferenceSample/2(Duration)  "<Duration>"
  RobotState/1 -> StateSelect/1
  BasePlan/1 -> PlanSelect/1
  PlanSelect/2 -> ReferenceSample/4(RefPose)  "<RefPose>"

== system homeMobileManipulator/MobileManipulator/MobileBase/PathPlanning ==
  RobotState : Inport  OutDataTypeStr=Bus: RobotState  LatchByDelayingOutsideSignal=on
  GoalPose : Inport  Port=2  PortDimensions=3  LatchByDelayingOutsideSignal=on
  CarriedExtent : Inport  Port=3  PortDimensions=3  LatchByDelayingOutsideSignal=on
  AltGoalPose : Inport  Port=4
  Request : TriggerPort  VariantControl=Variant  PortDimensions=1
  BasePathSearch : MATLAB Function  Description=SIMULINK-FIRST JUSTIFICATION: no dedicated block exists. Searched navlib with find_system('navlib','SearchDepth',2,'Type','Block'); Navigation Toolbox ships no planner block - plannerBiRRT, stateSpaceSE2, validatorOccupancyMap, pathmetrics and contopptraj are all System-object or function APIs. There is no native Simulink equivalent because a sampling-based search runs a data-dependent number of iterations with a growing tree; a fixed block diagram has no construct for it, so the native block count is undefined rather than merely over 15.  TreatAsAtomicUnit=on
  Grid : DataStoreRead  DataStoreName=NavMapGrid  IndexOptions=Index vector (dialog)  Indices=1  OutputSizes=1
  NextRequestId : Bias  Bias=1
  PlanTemplate : Constant  Value=basePlanInit  OutDataTypeStr=Bus: BasePlan
  RequestId : DataTypeConversion  OutDataTypeStr=uint32  SaturateOnIntegerOverflow=off  RndMeth=Floor
  RequestIdState : UnitDelay  SampleTime=-1
  StateSelect : BusSelector  OutputSignals=BasePose,Timestamp
  BasePlan : Outport  OutDataTypeStr=Bus: BasePlan  InitialOutput=basePlanInit
  wires:
  BasePathSearch/1(bplan) -> BasePlan/1
  AltGoalPose/1 -> BasePathSearch/8(altGoalPose)
  RequestId/1 -> RequestIdState/1, BasePathSearch/5(requestId)
  StateSelect/1 -> BasePathSearch/2(startPose)  "<BasePose>"
  PlanTemplate/1 -> BasePathSearch/7(planTemplate)
  Grid/1 -> BasePathSearch/1(gridMatrix)
  CarriedExtent/1 -> BasePathSearch/4(carriedExtent)
  StateSelect/2 -> BasePathSearch/6(simTime)  "<Timestamp>"
  RequestIdState/1 -> NextRequestId/1
  RobotState/1 -> StateSelect/1
  NextRequestId/1 -> RequestId/1  "NextRequestId"
  GoalPose/1 -> BasePathSearch/3(goalPose)

== system homeMobileManipulator/MobileManipulator/Plant/ArmKinematics ==
  ArmJointCmd : Inport
  JointError : Sum  Inputs=+-
  JointIntegrator : Integrator  InitialCondition=cfg.arm.stowConfig'
  JointLimit : Saturate  UpperLimit=armJointLimits(:,2)  LowerLimit=armJointLimits(:,1)
  JointRateLimit : Saturate  UpperLimit=cfg.arm.jointVelMax'  LowerLimit=-cfg.arm.jointVelMax'
  JointServoGain : Gain  Gain=1/cfg.arm.jointTimeConst
  ArmJointPos : Outport
  ArmJointVel : Outport  Port=2
  wires:
  JointLimit/1 -> JointError/1  "ArmJointCmdLimited"
  JointIntegrator/1 -> JointError/2, ArmJointPos/1  "ArmJointPos"
  ArmJointCmd/1 -> JointLimit/1
  JointError/1 -> JointServoGain/1  "JointError"
  JointRateLimit/1 -> JointIntegrator/1, ArmJointVel/1  "ArmJointVel"
  JointServoGain/1 -> JointRateLimit/1  "JointServoGain"

== system homeMobileManipulator/MobileManipulator/Plant/BaseKinematics ==
  BaseVelCmd : Inport
  PoseIntegration : Subsystem
  WheelKinematics : Subsystem
  BasePose : Outport
  BaseTwist : Outport  Port=2
  WheelSpeeds : Outport  Port=3
  wires:
  PoseIntegration/1(BasePose) -> BasePose/1  "BasePose"
  WheelKinematics/2(TwistRealised) -> PoseIntegration/1(TwistRealised), BaseTwist/1
  WheelKinematics/1(WheelSpeeds) -> WheelSpeeds/1  "WheelSpeeds"
  BaseVelCmd/1 -> WheelKinematics/1(TwistCmd)

== system homeMobileManipulator/MobileManipulator/Plant/CameraRig ==
  RobotConfig : Inport
  Enable : EnablePort
  CameraFrameArray : Concatenate  NumInputs=5
  Camera_1 : Subsystem
  Camera_2 : Subsystem
  Camera_3 : Subsystem
  Camera_4 : Subsystem
  WristCamera : Subsystem  Description=Wrist camera stream, CameraFrame index cfg.camera.wrist.index (5). Sixteen blocks rather than the ~15 guideline, and the six that push it over cannot be grouped away. This camera has no calibrated depth path: Simulation 3D Ray Tracer takes its ray origins and directions from dialog parameters, not from input ports, so it cannot follow a moving wrist. The frame therefore reports DepthSource = SOURCE_RENDER and must still fill the nested Calib (Bus: RayHits) element with an all-invalid value, which costs five typed Constants plus a Bus Creator. A single Constant holding invalidRayHits is the obvious one-block form and it does NOT work: Vector Concatenate in CameraRig/CameraFrameArray rejects the resulting frame even after every Bus Creator in the model was switched to InheritFromInputs = off. Nesting the six blocks in a subsystem was also tried and also rejected (a nested Bus Creator crossing an Outport will not concatenate against a flat one). The flat Bus Creator form is the only one that compiles and it is what the four fixed cameras use, so it stays flat here too. WristMountPose is the one part of this block that could be hidden, and it is.
  CameraFrames : Outport
  wires:
  Camera_4/1(CameraFrame) -> CameraFrameArray/4  "Frame_4"
  Camera_3/1(CameraFrame) -> CameraFrameArray/3  "Frame_3"
  CameraFrameArray/1 -> CameraFrames/1
  Camera_2/1(CameraFrame) -> CameraFrameArray/2  "Frame_2"
  WristCamera/1(CameraFrame) -> CameraFrameArray/5  "Frame_5"
  Camera_1/1(CameraFrame) -> CameraFrameArray/1  "Frame_1"
  RobotConfig/1 -> WristCamera/1(RobotConfig)

== system homeMobileManipulator/MobileManipulator/Plant/ChaseCamera ==
  RobotConfig : Inport
  Enable : EnablePort
  ChaseBoom : MATLAB Function  TreatAsAtomicUnit=on  SystemSampleTime=cfg.rates.scene
  ChaseCam : sim3dcameralib/Simulation 3D Camera  Priority=1  sensorTag=Sim3dSensor�  sensorId=26  sensorName=Sim3dSensor�  vehTagList={'ApartmentShell';'Custom ...';'HomeMobileManipulator';'Scene Origin';'SceneProps'}  vehTag=Custom ...  parentTag=HomeMobileManipulator  CoordinateSystem=Default  mountLoc=Origin  offsetFlag=on  tmountOffset=[0, 0, 0]  extTmount=on  rmountOffset=[0, 0, 0]  extRmount=on  FocalLength=cfg.view.chase.focalLength  OpticalCenter=cfg.view.chase.opticalCenter  ImageSize=cfg.view.chase.imageSize  RadialDistortion=[0, 0]  TangentialDistortion=[0, 0]  SensorSkew=0  VisualizeFieldOfView=off  FieldOfViewRange=61  DepthOutportEnabled=off  SemanticOutportEnabled=off  TransformOutportEnabled=on  SampleTime=cfg.rates.scene  mountPoint=[0 0 0]  mountOrientation=[0 0 0]  aMode=aMode  ID=26
  ChaseToEuler : robotcorelib/Coordinate Transformation Conversion  InputRepresentation=Homogeneous Transformation  InputEulerSequence=ZYX  ShowTrVecInputPort=on  OutputRepresentation=Euler Angles  OutputEulerSequence=ZYX  ShowTrVecOutputPort=on  SimulateUsing=Code generation
  ChaseView : VideoViewer  colormapValue=gray(256)  FigPos=[1087 792 570 522]  OpenAtMdlStart=off
  ChassisPose : robotmaniplib/Get Transform  RigidBodyTree=robot  SourceBody=chassis_link  TargetBody=map  SimulateUsing=Code generation
  RotToUnreal : Gain  Gain=[0 0 -1; 0 -1 0; 1 0 0]  Multiplication=Matrix(K*u)
  RotationRow : Reshape  OutputDimensionality=Row vector (2-D)
  TranslationRow : Reshape  OutputDimensionality=Row vector (2-D)
  Unused2 : Terminator
  Unused3 : Terminator
  wires:
  ChaseCam/3 -> Unused3/1
  ChaseCam/2 -> Unused2/1
  ChaseCam/1 -> ChaseView/1
  RotationRow/1 -> ChaseCam/2
  TranslationRow/1 -> ChaseCam/1
  ChaseToEuler/2 -> TranslationRow/1
  RotToUnreal/1 -> RotationRow/1
  ChaseToEuler/1 -> RotToUnreal/1
  ChaseBoom/1(T) -> ChaseToEuler/1
  ChassisPose/1 -> ChaseBoom/1(Tchassis)
  RobotConfig/1 -> ChassisPose/1

== system homeMobileManipulator/MobileManipulator/Plant/GraspCaptureGate ==
  GraspRequest : Inport
  AchievedAperture : Inport  Port=2
  GraspFramePos : Inport  Port=3
  GraspCandidate : Inport  Port=4
  ActorNameLookup : Subsystem  Description=|
      | SIMULATION 3D ROBOT'S TargetActor INPUT TAKES A NAME, NOT AN ID - and this model used to put an id on it.
      | 
      | robotics.slsim3d.internal.util.TargetGraspUtils.processTargetActorInput reads a SCALAR uint8 as "this input is disabled" and returns an empty name; Simulation3DRobotBlock.stepImpl then reports isTargetGrasped = false and returns before the grasp is considered at all. GraspCandidate.ActorId is a scalar uint8 and cfg.actor.noneId is uint8(0), so every value this model could put on that port was discarded. All four capture conditions held for 2.84 s and the mug never attached: no warning, no error, a well-formed false.
      | 
      | What the port wants is a uint8 ROW that char() turns into the actor's name, looked up as world.Actors.(name). hmmActorNames pads every actor name to cfg.actor.nameWidth characters so that a fixed-width Simulink signal and a struct-field lookup can agree - the block does no trimming, and world.Actors.('Mug_Red   ') is not world.Actors.Mug_Red. Row k of actorNameTable is registry ActorId k, because both are built from the same manifest in the same order.
      | 
      | The id still leaves this subsystem as TargetActorId, which is what AttachedActorId reports. This is the plant addressing the renderer, not perception naming an object: association stays geometric.
  CandidateSelect : BusSelector  OutputSignals=ActorId,Position,Extent,NumInCapture,Valid
  ExtentMatch : Subsystem
  GraspAuthorised : Logic  Inputs=4  IconShape=distinctive  AllPortsSameDT=off  OutDataTypeStr=boolean
  GraspHold : Subsystem  Description=|
      | CAPTURE IS A MOMENT, HOLDING IS A STATE.
      | 
      | GraspAuthorised conjoins four capture conditions, and one of them - WithinCapture - measures the grasp frame against the candidate position perception reconstructed ONCE, which does not move when the object does. Sent straight to the plant that released the object the instant it left the surface: LiftObject retreats cfg.sup.approachDepth = 0.12 m, nearly twice cfg.grasp.captureRadius = 0.0625 m, so InCapture went false and Simulation 3D Robot detached mid-lift.
      | 
      | The latch makes the plant's grasp mean what a gripper means: it closes when the capture conditions are met, and it lets go when it is TOLD to - not when the object it is already holding stops being where it used to be. GraspRequest is the only reset, so opening the jaws is what releases.
      | 
      | HeldPrev is a Unit Delay and not an S-R block because the reset has to win in the same step: AND(GraspRequest, OR(authorised, held)) is false the step GraspRequest falls, with no race between two edges.
  NoActor : Constant  Value=cfg.actor.noneId  OutDataTypeStr=uint8
  TargetActorSelect : Switch  Criteria=u2 ~= 0
  WithinCapture : Subsystem
  TargetActorId : Outport
  ActivateGrasp : Outport  Port=2
  TargetActorName : Outport  Port=3
  wires:
  TargetActorSelect/1 -> TargetActorId/1
  GraspHold/1(Holding) -> ActivateGrasp/1, TargetActorSelect/2  "ActivateGrasp"
  NoActor/1 -> TargetActorSelect/3
  GraspAuthorised/1 -> GraspHold/2(CaptureAuthorised)  "CaptureAuthorised"
  ExtentMatch/1(Match) -> GraspAuthorised/4
  WithinCapture/1(InCapture) -> GraspAuthorised/3  "InCapture"
  GraspRequest/1 -> GraspHold/1(GraspRequest), GraspAuthorised/1
  ActorNameLookup/1(ActorName) -> TargetActorName/1  "TargetActorName"
  CandidateSelect/4 -> WithinCapture/3(NumInCapture)  "<NumInCapture>"
  CandidateSelect/5 -> GraspAuthorised/2  "<Valid>"
  CandidateSelect/3 -> ExtentMatch/2(CandidateExtent)  "<Extent>"
  CandidateSelect/2 -> WithinCapture/2(CandidatePosition)  "<Position>"
  AchievedAperture/1 -> ExtentMatch/1(AchievedAperture)
  CandidateSelect/1 -> ActorNameLookup/1(ActorId), TargetActorSelect/1  "<ActorId>"
  GraspFramePos/1 -> WithinCapture/1(GraspFramePos)
  GraspCandidate/1 -> CandidateSelect/1
